simulink model "gm_soc_dlmc_rfsoc_zcu111"  (R2025b)
settings: Solver=FixedStepDiscrete  StartTime=0.0  StopTime=1e-3  RelTol=1e-3
PreLoadFcn:
  | soc_dlmc_rfsoc_init;
InitFcn:
  | soc_dlmc_rfsoc_init;
model workspace (MAT data in the model file):
  incrScale = 100
undefined symbols (not defined in the file or in its folder): Fs, I, Q, sampleTimeDL
libraries: hdlsllib x4, simulink x3, xilinxrfsoclib x1, dlhdlsim x1
settings Model: ModifiedByFormat=The MathWorks, Inc.  Creator=The MathWorks, Inc.  LastModifiedBy=The MathWorks, Inc.
settings SolverCC: PositivePriorityOrder=on
settings OptimizationCC: BlockReduction=off  ConditionallyExecuteInputs=off  DefaultParameterBehavior=Inlined  InheritOutputTypeSmallerThanSingle=on  EnhancedBackFolding=on  PassReuseOutputArgsAs=Individual arguments  ZeroExternalMemoryAtStartup=off  ZeroInternalMemoryAtStartup=off  MaxStackSize=64  OptimizeBlockOrder=speed  DifferentSizesBufferReuse=on  OptimizationCustomize=off  EfficientTunableParamExpr=on
settings DebuggingCC: ArtificialAlgebraicLoopMsg=error  UnderspecifiedInitializationDetection=Classic  MergeDetectMultiDrivingBlocksExec=none  SingleTaskRateTransMsg=warning  ParameterTunabilityLossMsg=error
settings HardwareCC: ProdBitPerPointer=32.0  ProdBitPerSizeT=32.0  ProdBitPerPtrDiffT=32.0  ProdLargestAtomicFloat=None  ProdIntDivRoundTo=Undefined  ProdEndianess=Unspecified  ProdWordSize=32.0  ProdHWDeviceType=ASIC/FPGA->ASIC/FPGA  TargetBitPerPointer=64.0  TargetBitPerSizeT=64.0  TargetBitPerPtrDiffT=64.0  TargetLongLongMode=on  TargetIntDivRoundTo=Zero  TargetEndianess=LittleEndian  TargetWordSize=64.0  TargetHWDeviceType=Custom Processor->MATLAB Host Computer  ProdEqTarget=off  HardwareBoardFeatureSet=SoCBlockset
settings ModelReferenceCC: ModelReferenceNumInstancesAllowed=Single  PropagateSignalLabelsOutOfModel=off
settings RTWCC: SystemTargetFile=ert.tlc  HardwareBoard=Xilinx Zynq UltraScale+ RFSoC ZCU111 Evaluation Kit  TLCOptions="-aInlineSetEventsForThisBaseRateFcn=TLC_FALSE -aSuppressMultiTaskScheduler=TLC_FALSE  -aRateBasedStepFcn=0"  TemplateMakefile=ert_default_tmf  Toolchain=Linaro AArch64 Linux v6.3.1  Description=Embedded Coder
settings CodeAppCC: ForceParamTrailComments=on  IgnoreCustomStorageClasses=off  OperatorAnnotations=on  SimulinkDataObjDesc=on  SFDataObjDesc=on  InsertBlockDesc=on
settings ERTTargetCC: SubcomponentCodeInterfacePackaging=Nonreusable function

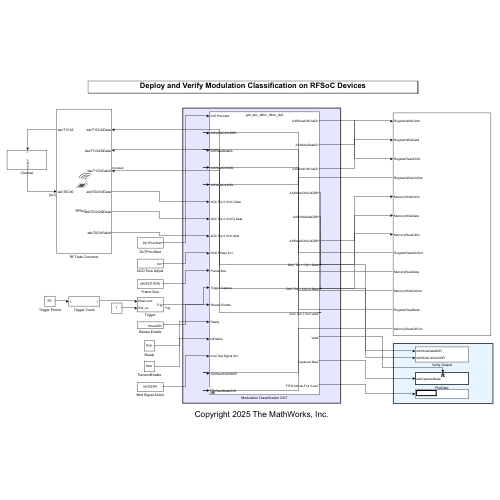
[thumbnail: Simulink's stored preview of the top-level diagram]
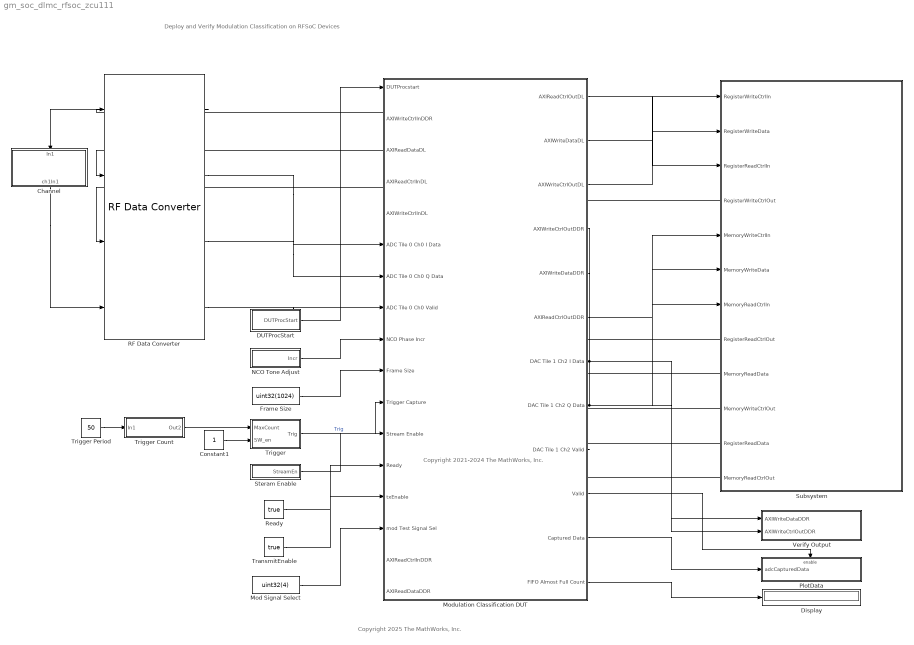
== system gm_soc_dlmc_rfsoc_zcu111 ==
  note: Copyright 2025 The MathWorks, Inc.
  note: Copyright 2021-2024 The MathWorks, Inc.
  note: Deploy and Verify Modulation Classification on RFSoC Devices
  Channel : Subsystem
      settings: PortSchema="{\"entries\":[{\"content\":{\"sides\":[{\"content\":{},\"type\":\"ConnectorPlacement.EquallySpacedRectSide\",\"uuid\":\"d9f03ac7-630b-4c9d-b2b7-0d7b8c069e33\"},{\"content\":{\"side\":\"RIGHT\"},\"type\":\"ConnectorPlacement.EquallySpacedRectSide\",\"uuid\":\"51f4549d-5d02-491e-ad49-36f7e9a624df\"},{\"content\":{\"connectorIds\":[\"In1\"],\"side\":\"TOP\"},\"type\":\"ConnectorPlacement.EquallySpacedRectSide\",\"uuid\":\"082c6092-c8df-4d99-92e1-0bd3b739b11a\"},{\"content\":{\"connectorIds\":[\"Out1\"],\"side\":\"BOTTOM\"},\"type\":\"ConnectorPlacement.EquallySpacedRectSide\",\"uuid\":\"6dad05eb-a37c-4890-a6f3-fc75ecfdc562\"}]},\"type\":\"ConnectorPlacement.EquallySpacedConnector\",\"uuid\":\"4d313c6e-a11a-46dc-b4b5-73957280d887\"}],\"packageUris\":[\"http://schema.mathworks.com/mf0/Connector/R2020b\"],\"version\":\"1.0\"}"
  Constant1 : Constant  OutDataTypeStr=boolean  SampleTime=-1
  DUTProcStart : Subsystem
  Display : Display
  Frame Size : Constant  Value=uint32(1024)  SampleTime=sampleTimeDL
  Mod Signal Select : Constant  Value=uint32(4)  SampleTime=-1
  Modulation Classification DUT : Subsystem  Variant=on  VariantControlMode=label  LabelModeActiveChoice=HDLC_internal_variant_GeneratedDUT
  NCO Tone Adjust : Subsystem
  PlotData : Subsystem
  RF Data Converter : xilinxrfsoclib/RF Data Converter  RFDCSim=Pass-through  tabPromptsCB=0  RFInterface=Customize  digitalInterface=I/Q  dac11Enable=off  dac12Enable=off  dac13Enable=off  dac14Enable=off  dac21Enable=off  dac22Enable=off  dac23Enable=on  dac24Enable=off  dac31Enable=off  dac32Enable=off  dac33Enable=off  dac34Enable=off  dac41Enable=off  dac42Enable=off  dac43Enable=off  dac44Enable=off  matchDACParam=on  dacSampleRate=2048  dacDatapathMode=Full Nyquist (0 to Fs/2)  interpolationMode=8  dacSamplesPerCycle=1  dacMixerType=Fine  dacMixerMode=I/Q->Real  dacMixerFrequency=Fs/2  dacNCOFrequency=0.5  dacNCOPhase=0  invertSyncFilter=off  dacTile1SampleRate=1000  dac11DatapathMode=Full Nyquist (0 to Fs/2)  dac11InterpolationMode=2  dac11SamplesPerCycle=2  dac11MixerType=Coarse  dac11MixerMode=I/Q->Real  dac11MixerFrequency=Fs/2  dac11NCOFrequency=0  dac11NCOPhase=0  dac11InvertSyncFilter=off  dac12DatapathMode=Full Nyquist (0 to Fs/2)  dac12InterpolationMode=2  dac12SamplesPerCycle=2  dac12MixerType=Coarse  dac12MixerMode=I/Q->Real  dac12MixerFrequency=Fs/2  dac12NCOFrequency=0  dac12NCOPhase=0  dac12InvertSyncFilter=off  dac13DatapathMode=Full Nyquist (0 to Fs/2)  dac13InterpolationMode=2  dac13SamplesPerCycle=2  dac13MixerType=Coarse  dac13MixerMode=I/Q->Real  dac13MixerFrequency=Fs/2  dac13NCOFrequency=0  dac13NCOPhase=0  dac13InvertSyncFilter=off  dac14DatapathMode=Full Nyquist (0 to Fs/2)  dac14InterpolationMode=2  dac14SamplesPerCycle=2  dac14MixerType=Coarse  dac14MixerMode=I/Q->Real  dac14MixerFrequency=Fs/2  dac14NCOFrequency=0  dac14NCOPhase=0  dac14InvertSyncFilter=off  dacTile2SampleRate=1000  dac21DatapathMode=Full Nyquist (0 to Fs/2)  dac21InterpolationMode=2  dac21SamplesPerCycle=2  dac21MixerType=Coarse  dac21MixerMode=I/Q->Real  dac21MixerFrequency=Fs/2  dac21NCOFrequency=0  dac21NCOPhase=0  dac21InvertSyncFilter=off  dac22DatapathMode=Full Nyquist (0 to Fs/2)  dac22InterpolationMode=2  dac22SamplesPerCycle=2  dac22MixerType=Coarse  dac22MixerMode=I/Q->Real  dac22MixerFrequency=Fs/2  dac22NCOFrequency=0  dac22NCOPhase=0  dac22InvertSyncFilter=off  dac23DatapathMode=Full Nyquist (0 to Fs/2)  dac23InterpolationMode=2  dac23SamplesPerCycle=2  dac23MixerType=Coarse  dac23MixerMode=I/Q->Real  dac23MixerFrequency=Fs/2  dac23NCOFrequency=0  dac23NCOPhase=0  dac23InvertSyncFilter=off  dac24DatapathMode=Full Nyquist (0 to Fs/2)  dac24InterpolationMode=2  dac24SamplesPerCycle=2  dac24MixerType=Coarse  dac24MixerMode=I/Q->Real  dac24MixerFrequency=Fs/2  dac24NCOFrequency=0  dac24NCOPhase=0  dac24InvertSyncFilter=off  dacTile3SampleRate=1000  dac31DatapathMode=Full Nyquist (0 to Fs/2)  dac31InterpolationMode=2  dac31SamplesPerCycle=2  dac31MixerType=Coarse  dac31MixerMode=I/Q->Real  dac31MixerFrequency=Fs/2  dac31NCOFrequency=0  dac31NCOPhase=0  dac31InvertSyncFilter=off  dac32DatapathMode=Full Nyquist (0 to Fs/2)  dac32InterpolationMode=2  dac32SamplesPerCycle=2  dac32MixerType=Coarse  dac32MixerMode=I/Q->Real  dac32MixerFrequency=Fs/2  dac32NCOFrequency=0  dac32NCOPhase=0  dac32InvertSyncFilter=off  dac33DatapathMode=Full Nyquist (0 to Fs/2)  dac33InterpolationMode=2  dac33SamplesPerCycle=2  dac33MixerType=Coarse  dac33MixerMode=I/Q->Real  dac33MixerFrequency=Fs/2  dac33NCOFrequency=0  dac33NCOPhase=0  dac33InvertSyncFilter=off  dac34DatapathMode=Full Nyquist (0 to Fs/2)  dac34InterpolationMode=2  dac34SamplesPerCycle=2  dac34MixerType=Coarse  dac34MixerMode=I/Q->Real  dac34MixerFrequency=Fs/2  dac34NCOFrequency=0  dac34NCOPhase=0  dac34InvertSyncFilter=off  dacTile4SampleRate=1000  dac41DatapathMode=Full Nyquist (0 to Fs/2)  dac41InterpolationMode=2  dac41SamplesPerCycle=2  dac41MixerType=Coarse  dac41MixerMode=I/Q->Real  dac41MixerFrequency=Fs/2  dac41NCOFrequency=0  dac41NCOPhase=0  dac41InvertSyncFilter=off  dac42DatapathMode=Full Nyquist (0 to Fs/2)  dac42InterpolationMode=2  dac42SamplesPerCycle=2  dac42MixerType=Coarse  dac42MixerMode=I/Q->Real  dac42MixerFrequency=Fs/2  dac42NCOFrequency=0  dac42NCOPhase=0  dac42InvertSyncFilter=off  dac43DatapathMode=Full Nyquist (0 to Fs/2)  dac43InterpolationMode=2  dac43SamplesPerCycle=2  dac43MixerType=Coarse  dac43MixerMode=I/Q->Real  dac43MixerFrequency=Fs/2  dac43NCOFrequency=0  dac43NCOPhase=0  dac43InvertSyncFilter=off  dac44DatapathMode=Full Nyquist (0 to Fs/2)  dac44InterpolationMode=2  dac44SamplesPerCycle=2  dac44MixerType=Coarse  dac44MixerMode=I/Q->Real  dac44MixerFrequency=Fs/2  dac44NCOFrequency=0  dac44NCOPhase=0  dac44InvertSyncFilter=off  adc11Enable=on  adc12Enable=off  adc13Enable=off  adc14Enable=off  adc21Enable=off  adc22Enable=off  adc23Enable=off  adc24Enable=off  adc31Enable=off  adc32Enable=off  adc33Enable=off  adc34Enable=off  adc41Enable=off  adc42Enable=off  adc43Enable=off  adc44Enable=off  adcOutUnpackedData=on  matchADCParam=on  adcSampleRate=2048  decimationMode=8  adcSamplesPerCycle=1  adcMixerType=Fine  adcMixerMode=Real->I/Q  adcMixerFrequency=Fs/2  adcNCOFrequency=-0.5  adcNCOPhase=0  adcTile1SampleRate=1000  adc11DecimationMode=2  adc11SamplesPerCycle=2  adc11MixerType=Coarse  adc11MixerMode=Real->I/Q  adc11MixerFrequency=Fs/2  adc11NCOFrequency=0  adc11NCOPhase=0  adc12DecimationMode=2  adc12SamplesPerCycle=2  adc12MixerType=Coarse  adc12MixerMode=Real->I/Q  adc12MixerFrequency=Fs/2  adc12NCOFrequency=0  adc12NCOPhase=0  adc13DecimationMode=2  adc13SamplesPerCycle=2  adc13MixerType=Coarse  adc13MixerMode=Real->I/Q  adc13MixerFrequency=Fs/2  adc13NCOFrequency=0  adc13NCOPhase=0  adc14DecimationMode=2  adc14SamplesPerCycle=2  adc14MixerType=Coarse  adc14MixerMode=Real->I/Q  adc14MixerFrequency=Fs/2  adc14NCOFrequency=0  adc14NCOPhase=0  adcTile2SampleRate=1000  adc21DecimationMode=2  adc21SamplesPerCycle=2  adc21MixerType=Coarse  adc21MixerMode=Real->I/Q  adc21MixerFrequency=Fs/2  adc21NCOFrequency=0  adc21NCOPhase=0  adc22DecimationMode=2  adc22SamplesPerCycle=2  adc22MixerType=Coarse  adc22MixerMode=Real->I/Q  adc22MixerFrequency=Fs/2  adc22NCOFrequency=0  adc22NCOPhase=0  adc23DecimationMode=2  adc23SamplesPerCycle=2  adc23MixerType=Coarse  adc23MixerMode=Real->I/Q  adc23MixerFrequency=Fs/2  adc23NCOFrequency=0  adc23NCOPhase=0  adc24DecimationMode=2  adc24SamplesPerCycle=2  adc24MixerType=Coarse  adc24MixerMode=Real->I/Q  adc24MixerFrequency=Fs/2  adc24NCOFrequency=0  adc24NCOPhase=0  adcTile3SampleRate=1000  adc31DecimationMode=2  adc31SamplesPerCycle=2  adc31MixerType=Coarse  adc31MixerMode=Real->I/Q  adc31MixerFrequency=Fs/2  adc31NCOFrequency=0  adc31NCOPhase=0  adc32DecimationMode=2  adc32SamplesPerCycle=2  adc32MixerType=Coarse  adc32MixerMode=Real->I/Q  adc32MixerFrequency=Fs/2  adc32NCOFrequency=0  adc32NCOPhase=0  adc33DecimationMode=2  adc33SamplesPerCycle=2  adc33MixerType=Coarse  adc33MixerMode=Real->I/Q  adc33MixerFrequency=Fs/2  adc33NCOFrequency=0  adc33NCOPhase=0  adc34DecimationMode=2  adc34SamplesPerCycle=2  adc34MixerType=Coarse  adc34MixerMode=Real->I/Q  adc34MixerFrequency=Fs/2  adc34NCOFrequency=0  adc34NCOPhase=0  adcTile4SampleRate=1000  adc41DecimationMode=2  adc41SamplesPerCycle=2  adc41MixerType=Coarse  adc41MixerMode=Real->I/Q  adc41MixerFrequency=Fs/2  adc41NCOFrequency=0  adc41NCOPhase=0  adc42DecimationMode=2  adc42SamplesPerCycle=2  adc42MixerType=Coarse  adc42MixerMode=Real->I/Q  adc42MixerFrequency=Fs/2  adc42NCOFrequency=0  adc42NCOPhase=0  adc43DecimationMode=2  adc43SamplesPerCycle=2  adc43MixerType=Coarse  adc43MixerMode=Real->I/Q  adc43MixerFrequency=Fs/2  adc43NCOFrequency=0  adc43NCOPhase=0  adc44DecimationMode=2  adc44SamplesPerCycle=2  adc44MixerType=Coarse  adc44MixerMode=Real->I/Q  adc44MixerFrequency=Fs/2  adc44NCOFrequency=0  adc44NCOPhase=0  multiTileSync=off  externalPLL=off  dacRealTimeNCOPortsEnable=off  adcRealTimeNCOPortsEnable=off  adcRealTimePortsEnable=off  adcThresholdMode=Sticky over  adcThreshold1=0  adcDelayCounter=0  adcThreshold2Mode=Sticky over  adcThreshold2=0  adcThreshold2DelayCounter=0  adc11ThresholdMode=Sticky over  adc11Threshold1=0  adc11DelayCounter=0  adc11Threshold2Mode=Sticky over  adc11Threshold2=0  adc11Threshold2DelayCounter=0  adc12ThresholdMode=Sticky over  adc12Threshold1=0  adc12DelayCounter=0  adc12Threshold2Mode=Sticky over  adc12Threshold2=0  adc12Threshold2DelayCounter=0  adc13ThresholdMode=Sticky over  adc13Threshold1=0  adc13DelayCounter=0  adc13Threshold2Mode=Sticky over  adc13Threshold2=0  adc13Threshold2DelayCounter=0  adc14ThresholdMode=Sticky over  adc14Threshold1=0  adc14DelayCounter=0  adc14Threshold2Mode=Sticky over  adc14Threshold2=0  adc14Threshold2DelayCounter=0  adc21ThresholdMode=Sticky over  adc21Threshold1=0  adc21DelayCounter=0  adc21Threshold2Mode=Sticky over  adc21Threshold2=0  adc21Threshold2DelayCounter=0  adc22ThresholdMode=Sticky over  adc22Threshold1=0  adc22DelayCounter=0  adc22Threshold2Mode=Sticky over  adc22Threshold2=0  adc22Threshold2DelayCounter=0  adc23ThresholdMode=Sticky over  adc23Threshold1=0  adc23DelayCounter=0  adc23Threshold2Mode=Sticky over  adc23Threshold2=0  adc23Threshold2DelayCounter=0  adc24ThresholdMode=Sticky over  adc24Threshold1=0  adc24DelayCounter=0  adc24Threshold2Mode=Sticky over  adc24Threshold2=0  adc24Threshold2DelayCounter=0  adc31ThresholdMode=Sticky over  adc31Threshold1=0  adc31DelayCounter=0  adc31Threshold2Mode=Sticky over  adc31Threshold2=0  adc31Threshold2DelayCounter=0  adc32ThresholdMode=Sticky over  adc32Threshold1=0  adc32DelayCounter=0  adc32Threshold2Mode=Sticky over  adc32Threshold2=0  adc32Threshold2DelayCounter=0  adc33ThresholdMode=Sticky over  adc33Threshold1=0  adc33DelayCounter=0  adc33Threshold2Mode=Sticky over  adc33Threshold2=0  adc33Threshold2DelayCounter=0  adc34ThresholdMode=Sticky over  adc34Threshold1=0  adc34DelayCounter=0  adc34Threshold2Mode=Sticky over  adc34Threshold2=0  adc34Threshold2DelayCounter=0  adc41ThresholdMode=Sticky over  adc41Threshold1=0  adc41DelayCounter=0  adc41Threshold2Mode=Sticky over  adc41Threshold2=0  adc41Threshold2DelayCounter=0  adc42ThresholdMode=Sticky over  adc42Threshold1=0  adc42DelayCounter=0  adc42Threshold2Mode=Sticky over  adc42Threshold2=0  adc42Threshold2DelayCounter=0  adc43ThresholdMode=Sticky over  adc43Threshold1=0  adc43DelayCounter=0  adc43Threshold2Mode=Sticky over  adc43Threshold2=0  adc43Threshold2DelayCounter=0  adc44ThresholdMode=Sticky over  adc44Threshold1=0  adc44DelayCounter=0  adc44Threshold2Mode=Sticky over  adc44Threshold2=0  adc44Threshold2DelayCounter=0
      settings: LibrarySourceBlock=rfsoczcu111lib/RF Data Converter
  Ready : Constant  Value=true  OutDataTypeStr=boolean  SampleTime=sampleTimeDL
  Steram Enable : Subsystem
  Subsystem : Subsystem
      settings: PortSchema="{\"entries\":[{\"content\":{\"sides\":[{\"content\":{\"connectorIds\":[\"In1\",\"In2\",\"In3\",\"Out1\",\"In4\",\"In5\",\"In6\",\"Out2\",\"Out3\",\"Out4\",\"Out5\",\"Out6\"]},\"type\":\"ConnectorPlacement.EquallySpacedRectSide\",\"uuid\":\"5a4fc050-6ba1-453f-93c1-69d3faa6b955\"},{\"content\":{\"side\":\"RIGHT\"},\"type\":\"ConnectorPlacement.EquallySpacedRectSide\",\"uuid\":\"8677897f-1116-461c-9ed1-5f1d76ce8123\"},{\"content\":{\"side\":\"TOP\"},\"type\":\"ConnectorPlacement.EquallySpacedRectSide\",\"uuid\":\"ae99672c-8e60-4409-bdc4-49d2ca209157\"}]},\"type\":\"ConnectorPlacement.EquallySpacedConnector\",\"uuid\":\"10ae4214-cc16-400c-88d8-4466e97b849b\"}],\"packageUris\":[\"http://schema.mathworks.com/mf0/Connector/R2020b\"],\"version\":\"1.0\"}"
  TransmitEnable : Constant  Value=true  OutDataTypeStr=boolean  SampleTime=-1
  Trigger : Subsystem
  Trigger Count : Subsystem
  Trigger Period : Constant  Value=50  OutDataTypeStr=uint32  SampleTime=sampleTimeDL
  Verify Output : Subsystem
  wires:
  Trigger Count/1(Out2) -> Trigger/1(MaxCount)
  Constant1/1 -> Trigger/2(SW_en)
  Trigger Period/1 -> Trigger Count/1(In1)
  RF Data Converter/1 -> Channel/1(In1)
  Channel/1(ch1In1) -> RF Data Converter/4
  DUTProcStart/1(DUTProcStart) -> Modulation Classification DUT/1(DUTProcstart)
  Subsystem/4(MemoryWriteCtrlOut) -> Modulation Classification DUT/2(AXIWriteCtrlInDDR)
  Subsystem/5(RegisterReadData) -> Modulation Classification DUT/3(AXIReadDataDL)
  Subsystem/2(RegisterReadCtrlOut) -> Modulation Classification DUT/4(AXIReadCtrlInDL)
  Subsystem/1(RegisterWriteCtrlOut) -> Modulation Classification DUT/5(AXIWriteCtrlInDL)
  RF Data Converter/2 -> Modulation Classification DUT/6(ADC Tile 0 Ch0 I Data)
  RF Data Converter/3 -> Modulation Classification DUT/7(ADC Tile 0 Ch0 Q Data)
  RF Data Converter/4 -> Modulation Classification DUT/8(ADC Tile 0 Ch0 Valid)
  NCO Tone Adjust/1(Incr) -> Modulation Classification DUT/9(NCO Phase Incr)
  Frame Size/1 -> Modulation Classification DUT/10(Frame Size)
  Trigger/1(Trig) -> Modulation Classification DUT/11(Trigger Capture)  "Trig"
  Steram Enable/1(StreamEn) -> Modulation Classification DUT/12(Stream Enable)
  Ready/1 -> Modulation Classification DUT/13(Ready)
  TransmitEnable/1 -> Modulation Classification DUT/14(txEnable)
  Mod Signal Select/1 -> Modulation Classification DUT/15(mod Test Signal Sel)
  Subsystem/6(MemoryReadCtrlOut) -> Modulation Classification DUT/16(AXIReadCtrlInDDR)
  Subsystem/3(MemoryReadData) -> Modulation Classification DUT/17(AXIReadDataDDR)
  Modulation Classification DUT/1(AXIReadCtrlOutDL) -> Subsystem/3(RegisterReadCtrlIn)
  Modulation Classification DUT/2(AXIWriteDataDL) -> Subsystem/2(RegisterWriteData)
  Modulation Classification DUT/3(AXIWriteCtrlOutDL) -> Subsystem/1(RegisterWriteCtrlIn)
  Modulation Classification DUT/4(AXIWriteCtrlOutDDR) -> Verify Output/2(AXIWriteCtrlOutDDR), Subsystem/4(MemoryWriteCtrlIn)
  Modulation Classification DUT/5(AXIWriteDataDDR) -> Subsystem/5(MemoryWriteData), Verify Output/1(AXIWriteDataDDR)
  Modulation Classification DUT/6(AXIReadCtrlOutDDR) -> Subsystem/6(MemoryReadCtrlIn)
  Modulation Classification DUT/7(DAC Tile 1 Ch2 I Data) -> RF Data Converter/1
  Modulation Classification DUT/8(DAC Tile 1 Ch2 Q Data) -> RF Data Converter/2
  Modulation Classification DUT/9(DAC Tile 1 Ch2 Valid) -> RF Data Converter/3
  Modulation Classification DUT/10(Valid) -> PlotData/Enable
  Modulation Classification DUT/11(Captured Data) -> PlotData/1(adcCapturedData)
  Modulation Classification DUT/12(FIFO Almost Full Count) -> Display/1

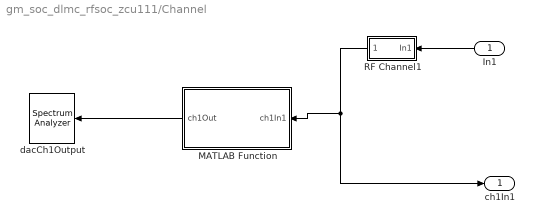
== system gm_soc_dlmc_rfsoc_zcu111/Channel ==
  In1 : Inport
  MATLAB Function : MATLAB Function  TreatAsAtomicUnit=on
  RF Channel1 : Subsystem
  dacCh1Output : SpectrumAnalyzer  WindowPosition=[553.000000,114.000000,800.000000,446.000000,]  ScopeFrameLocation=window  SampleRateSource=Property  SampleRate=256000000  Span=983040000  CenterFrequency=491520000  StartFrequency=0  StopFrequency=983040000  YLimits=[34.6843 100.6812]  SelectedToolstripTab=spectrumAnalyzerToolstrip.channelMeasurementsTab
  ch1In1 : Outport
  wires:
  RF Channel1/1(Out1) -> ch1In1/1, MATLAB Function/1(ch1In1)
  MATLAB Function/1(ch1Out) -> dacCh1Output/1
  In1/1 -> RF Channel1/1(In1)

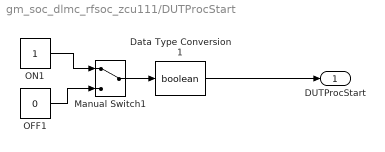
== system gm_soc_dlmc_rfsoc_zcu111/DUTProcStart ==
  Data Type Conversion1 : DataTypeConversion  OutDataTypeStr=boolean  SaturateOnIntegerOverflow=off  RndMeth=Floor
  Manual Switch1 : ManualSwitch
  OFF1 : Constant  Value=0  OutDataTypeStr=boolean  SampleTime=sampleTimeDL
  ON1 : Constant  OutDataTypeStr=boolean  SampleTime=sampleTimeDL
  DUTProcStart : Outport  VectorParamsAs1DForOutWhenUnconnected=off
  wires:
  Data Type Conversion1/1 -> DUTProcStart/1
  OFF1/1 -> Manual Switch1/2
  ON1/1 -> Manual Switch1/1
  Manual Switch1/1 -> Data Type Conversion1/1

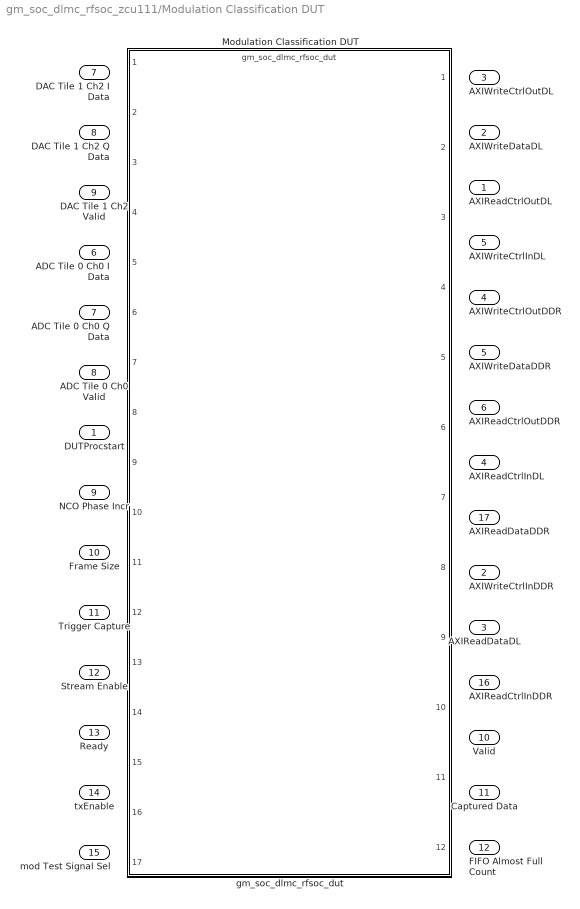
== system gm_soc_dlmc_rfsoc_zcu111/Modulation Classification DUT ==
  DUTProcstart : Inport
  AXIWriteCtrlInDDR : Inport  Port=2  OutDataTypeStr=Bus: BusAXIWriteCtrlS2M
  AXIReadDataDL : Inport  Port=3
  AXIReadCtrlInDL : Inport  Port=4  OutDataTypeStr=Bus: BusAXIReadCtrlS2M
  AXIWriteCtrlInDL : Inport  Port=5  OutDataTypeStr=Bus: BusAXIWriteCtrlS2M
  ADC Tile 0 Ch0 I Data : Inport  Port=6
  ADC Tile 0 Ch0 Q Data : Inport  Port=7
  ADC Tile 0 Ch0 Valid : Inport  Port=8
  NCO Phase Incr : Inport  Port=9
  Frame Size : Inport  Port=10
  Trigger Capture : Inport  Port=11
  Stream Enable : Inport  Port=12
  Ready : Inport  Port=13
  txEnable : Inport  Port=14
  mod Test Signal Sel : Inport  Port=15
  AXIReadCtrlInDDR : Inport  Port=16  OutDataTypeStr=Bus: BusAXIReadCtrlS2M
  AXIReadDataDDR : Inport  Port=17
  Modulation Classification DUT : ModelReference  ModelNameDialog=soc_dlmc_rfsoc_dut  SimulationMode=Normal  VariantControl=HDLC_internal_variant_OriginalDUT  ModelReferenceVersion=10.0
      settings: PortSchema="{\"entries\":[{\"content\":{\"sides\":[{\"content\":{\"connectorIds\":[\"Out7\",\"Out8\",\"Out9\",\"In6\",\"In7\",\"In8\",\"In1\",\"In9\",\"In10\",\"In11\",\"In12\",\"In13\",\"In14\",\"In15\"]},\"type\":\"ConnectorPlacement.EquallySpacedRectSide\",\"uuid\":\"df332c63-db3b-4cca-9e11-35333659716a\"},{\"content\":{\"connectorIds\":[\"Out3\",\"Out2\",\"Out1\",\"In5\",\"Out4\",\"Out5\",\"Out6\",\"In4\",\"In17\",\"In2\",\"In3\",\"In16\",\"Out10\",\"Out11\",\"Out12\"],\"side\":\"RIGHT\"},\"type\":\"ConnectorPlacement.EquallySpacedRectSide\",\"uuid\":\"c5d29afc-425e-406b-b67c-36cf7ce339ff\"},{\"content\":{\"side\":\"TOP\"},\"type\":\"ConnectorPlacement.EquallySpacedRectSide\",\"uuid\":\"3911ee3d-84ac-49ca-9a69-c94e8d017ed8\"}]},\"type\":\"ConnectorPlacement.EquallySpacedConnector\",\"uuid\":\"9d3b9653-3881-4eeb-b670-4519ee7519a2\"}],\"packageUris\":[\"http://schema.mathworks.com/mf0/Connector/R2020b\"],\"version\":\"1.0\"}"
  gm_soc_dlmc_rfsoc_dut : ModelReference  ModelNameDialog=gm_soc_dlmc_rfsoc_dut  SimulationMode=Normal  VariantControl=HDLC_internal_variant_GeneratedDUT  ModelReferenceVersion=10.1
  AXIReadCtrlOutDL : Outport  OutDataTypeStr=Bus: BusAXIReadCtrlM2S
  AXIWriteDataDL : Outport  Port=2
  AXIWriteCtrlOutDL : Outport  Port=3  OutDataTypeStr=Bus: BusAXIWriteCtrlM2S
  AXIWriteCtrlOutDDR : Outport  Port=4  OutDataTypeStr=Bus: BusAXIWriteCtrlM2S
  AXIWriteDataDDR : Outport  Port=5
  AXIReadCtrlOutDDR : Outport  Port=6  OutDataTypeStr=Bus: BusAXIReadCtrlM2S
  DAC Tile 1 Ch2 I Data : Outport  Port=7
  DAC Tile 1 Ch2 Q Data : Outport  Port=8
  DAC Tile 1 Ch2 Valid : Outport  Port=9
  Valid : Outport  Port=10
  Captured Data : Outport  Port=11
  FIFO Almost Full Count : Outport  Port=12

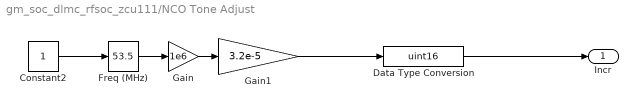
== system gm_soc_dlmc_rfsoc_zcu111/NCO Tone Adjust ==
  Constant2 : Constant  SampleTime=-1
  Data Type Conversion : DataTypeConversion  OutDataTypeStr=uint16  SaturateOnIntegerOverflow=off  RndMeth=Floor
  Freq (MHz) : simulink/Math Operations/Slider Gain  gain=53.5  low=0  high=250
  Gain : Gain  Gain=1e6
  Gain1 : Gain  Gain=3.2e-5
  Incr : Outport  VectorParamsAs1DForOutWhenUnconnected=off
  wires:
  Freq (MHz)/1 -> Gain/1
  Constant2/1 -> Freq (MHz)/1
  Data Type Conversion/1 -> Incr/1
  Gain1/1 -> Data Type Conversion/1
  Gain/1 -> Gain1/1

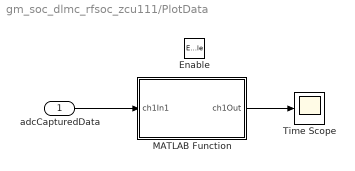
== system gm_soc_dlmc_rfsoc_zcu111/PlotData ==
  adcCapturedData : Inport
  Enable : EnablePort
  MATLAB Function : MATLAB Function  TreatAsAtomicUnit=on
  Time Scope : Scope
      settings: TimeUnits=Metric (based on Time Span)  ActiveDisplayYMinimum=-20141.25  ActiveDisplayYMaximum=20141.25  YLabel=Amplitude
  wires:
  MATLAB Function/1(ch1Out) -> Time Scope/1
  adcCapturedData/1 -> MATLAB Function/1(ch1In1)

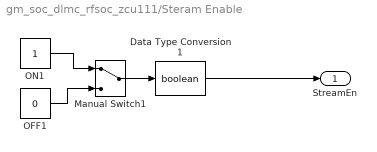
== system gm_soc_dlmc_rfsoc_zcu111/Steram Enable ==
  Data Type Conversion1 : DataTypeConversion  OutDataTypeStr=boolean  SaturateOnIntegerOverflow=off  RndMeth=Floor
  Manual Switch1 : ManualSwitch
  OFF1 : Constant  Value=0  OutDataTypeStr=boolean  SampleTime=sampleTimeDL
  ON1 : Constant  OutDataTypeStr=boolean  SampleTime=sampleTimeDL
  StreamEn : Outport  VectorParamsAs1DForOutWhenUnconnected=off
  wires:
  Data Type Conversion1/1 -> StreamEn/1
  OFF1/1 -> Manual Switch1/2
  ON1/1 -> Manual Switch1/1
  Manual Switch1/1 -> Data Type Conversion1/1

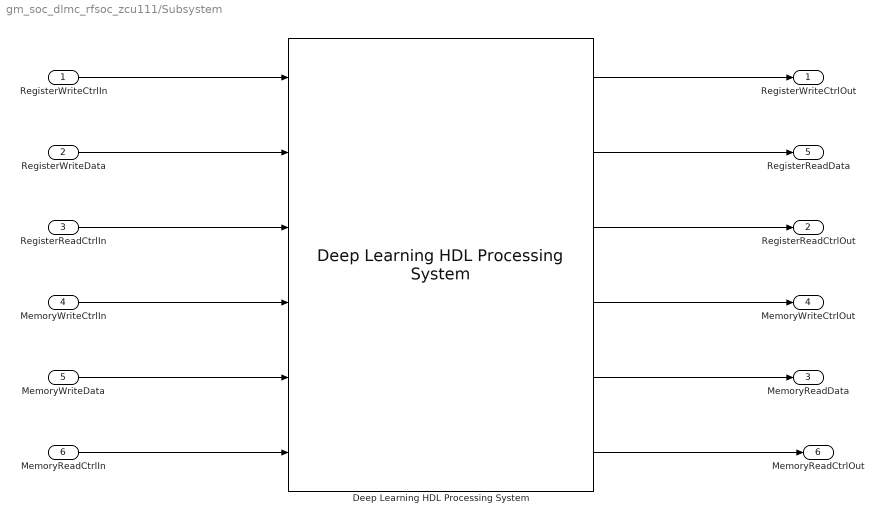
== system gm_soc_dlmc_rfsoc_zcu111/Subsystem ==
  RegisterWriteCtrlIn : Inport
  RegisterWriteData : Inport  Port=2
  RegisterReadCtrlIn : Inport  Port=3
  MemoryWriteCtrlIn : Inport  Port=4
  MemoryWriteData : Inport  Port=5
  MemoryReadCtrlIn : Inport  Port=6
  Deep Learning HDL Processing System : dlhdlsim/Deep Learning HDL Processing System  networkOption=Network from MAT-file  netFunction=getDigitsNetwork  netFile=dlhdltrainedModulationClassificationNetwork.mat  activationLayer=FC1  multiOutputs={''}  frameBufferCount=30  importExportOption=Import Processor Configuration from MATLAB function  importVar=helperGetProcessorConfig  exportVar=hPCInSimulink  convModuleGen=on  convLRNBlockGeneration=off  convSegmentationBlockGeneration=on  convConvThreadNumber=9  convInputMemorySize=[227 227 3]  convOutputMemorySize=[227 227 3]  convFeatureSizeLimit=2048  fcModuleGen=on  fcSoftmaxBlockGeneration=off  fcFCThreadNumber=4  fcInputMemorySize=25088  fcOutputMemorySize=4096  customModuleGen=on  addModuleGen=on  multModuleGen=on  resizeModuleGen=off  sigmoidModuleGen=off  tanhModuleGen=off  mishModuleGen=off  swishModuleGen=off  customInputMemorySize=40  customOutputMemorySize=120  processingMode=register  runTimeControl=register  runTimeStatus=register  inputStreamControl=register  outputStreamControl=register  setupControl=register  processorDataType=single  UseVendorLibrary=on  exportRegAddr=on  Parameter35='Xilinx Zynq UltraScale+ MPSoC ZCU102 Evaluation Kit'  Parameter36=200  Parameter37='Xilinx Vivado'  Parameter38='AXI-Stream DDR Memory Access : 3-AXIM'  Parameter39='Zynq UltraScale+'  Parameter40='xczu9eg-ffvb1156-2-e'  Parameter41=''  Parameter42=''  singleToInt8Exp=1  int8ToSingleExp=-4  exporthPC=off  hPCInSimulink=hPCInSimulink  axiDataWordWidth=4  convThreadNumber=3  fcThreadNumber=4  dataTransferNumber=4  numOfPaddedInputChannels=4  networkInputSize="1  1024     2"  networkOutputSize=11  paddedOutputSize=12  convWeightBlockGeneration=off  convGELUBlockGeneration=off  fcGELUBlockGeneration=off
  RegisterWriteCtrlOut : Outport
  RegisterReadCtrlOut : Outport  Port=2
  MemoryReadData : Outport  Port=3
  MemoryWriteCtrlOut : Outport  Port=4
  RegisterReadData : Outport  Port=5
  MemoryReadCtrlOut : Outport  Port=6
  wires:
  Deep Learning HDL Processing System/6 -> MemoryReadCtrlOut/1
  Deep Learning HDL Processing System/5 -> MemoryReadData/1
  RegisterReadCtrlIn/1 -> Deep Learning HDL Processing System/3
  RegisterWriteCtrlIn/1 -> Deep Learning HDL Processing System/1
  RegisterWriteData/1 -> Deep Learning HDL Processing System/2
  MemoryWriteData/1 -> Deep Learning HDL Processing System/5
  MemoryReadCtrlIn/1 -> Deep Learning HDL Processing System/6
  Deep Learning HDL Processing System/2 -> RegisterReadData/1
  MemoryWriteCtrlIn/1 -> Deep Learning HDL Processing System/4
  Deep Learning HDL Processing System/4 -> MemoryWriteCtrlOut/1
  Deep Learning HDL Processing System/1 -> RegisterWriteCtrlOut/1
  Deep Learning HDL Processing System/3 -> RegisterReadCtrlOut/1

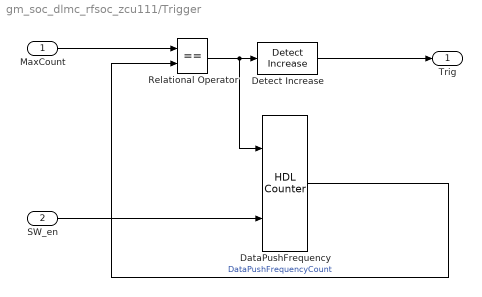
== system gm_soc_dlmc_rfsoc_zcu111/Trigger ==
  MaxCount : Inport
  SW_en : Inport  Port=2
  DataPushFrequency : hdlsllib/Sources/HDL Counter  CountType=Free running  CountInit=0  CountStep=1  CountMax=25  CountFromType=Initial value  CountFrom=0  CountResetPort=on  CountLoadPort=off  CountEnbPort=on  CountDirPort=off  CountHitOutputPort=off  CountDataType=Unsigned  CountWordLen=32  CountFracLen=0  CountSampTime=1
  Detect Increase : simulink/Logic and Bit Operations/Detect Increase  vinit=0.0  OutDataTypeStr=boolean
  Relational Operator : RelationalOperator  Operator===  OutDataTypeStr=boolean  RndMeth=Simplest  InputSameDT=off
  Trig : Outport  VectorParamsAs1DForOutWhenUnconnected=off
  wires:
  Relational Operator/1 -> DataPushFrequency/1, Detect Increase/1
  DataPushFrequency/1 -> Relational Operator/2  "DataPushFrequencyCount"
  Detect Increase/1 -> Trig/1
  SW_en/1 -> DataPushFrequency/2
  MaxCount/1 -> Relational Operator/1

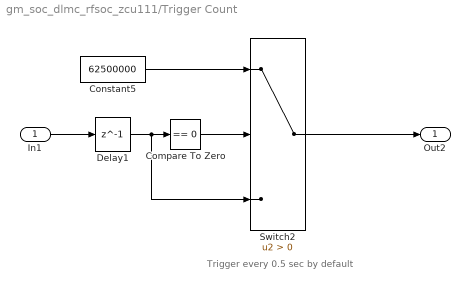
== system gm_soc_dlmc_rfsoc_zcu111/Trigger Count ==
  note: Trigger every 0.5 sec by default
  In1 : Inport
  Compare To Zero : simulink/Logic and Bit Operations/Compare To Zero  relop===  OutDataTypeStr=boolean
  Constant5 : Constant  Value=62500000  OutDataTypeStr=uint32  SampleTime=-1
  Delay1 : Delay  DelayLength=1
  Switch2 : Switch  Criteria=u2 > Threshold  SaturateOnIntegerOverflow=off  InputSameDT=off
  Out2 : Outport  VectorParamsAs1DForOutWhenUnconnected=off
  wires:
  In1/1 -> Delay1/1
  Constant5/1 -> Switch2/1
  Delay1/1 -> Switch2/3, Compare To Zero/1
  Switch2/1 -> Out2/1
  Compare To Zero/1 -> Switch2/2

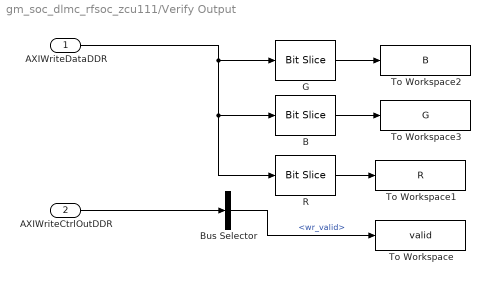
== system gm_soc_dlmc_rfsoc_zcu111/Verify Output ==
  AXIWriteDataDDR : Inport
  AXIWriteCtrlOutDDR : Inport  Port=2
  B : hdlsllib/Logic and Bit Operations/Bit Slice  lidx=63  ridx=32
  Bus Selector : BusSelector  OutputSignals=wr_valid
  G : hdlsllib/Logic and Bit Operations/Bit Slice  lidx=95  ridx=64
  R : hdlsllib/Logic and Bit Operations/Bit Slice  lidx=31  ridx=0
  To Workspace : ToWorkspace  VariableName=valid  SaveFormat=Timeseries  SampleTime=-1
  To Workspace1 : ToWorkspace  VariableName=R  SaveFormat=Timeseries  SampleTime=-1
  To Workspace2 : ToWorkspace  VariableName=B  SaveFormat=Timeseries  SampleTime=-1
  To Workspace3 : ToWorkspace  VariableName=G  SaveFormat=Timeseries  SampleTime=-1
  wires:
  Bus Selector/1 -> To Workspace/1  "<wr_valid>"
  AXIWriteCtrlOutDDR/1 -> Bus Selector/1
  R/1 -> To Workspace1/1
  B/1 -> To Workspace3/1
  G/1 -> To Workspace2/1
  AXIWriteDataDDR/1 -> R/1, B/1, G/1

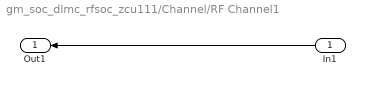
== system gm_soc_dlmc_rfsoc_zcu111/Channel/RF Channel1 ==
  In1 : Inport
  Out1 : Outport
  wires:
  In1/1 -> Out1/1

== matlab function gm_soc_dlmc_rfsoc_zcu111/PlotData/MATLAB Function ==
  data: ch1In1 input; ch1Out output size=1
function ch1Out  = fcn(ch1In1)

tmp = typecast(ch1In1, 'int16');
% iSamples = typecast(tmp(2), 'int16');
% qSamples = typecast(tmp(1), 'int16');
% ch1Out = complex(iSamples', qSamples');
ch1Out = complex(tmp(1), tmp(2));

end

== matlab function gm_soc_dlmc_rfsoc_zcu111/Channel/MATLAB Function ==
  data: ch1In1 input; ch1Out output size=1
function ch1Out  = fcn(ch1In1)

ch1Out = complex(ch1In1(1:2:end), ch1In1(2:2:end));

end
